simulink model "current_senzor"  (R2026a)
settings: Solver=VariableStepAuto
libraries: fl_lib x1, nesl_utility x1
settings Model: Creator=Fer Alexandru  LastModifiedBy=Fer Alexandru

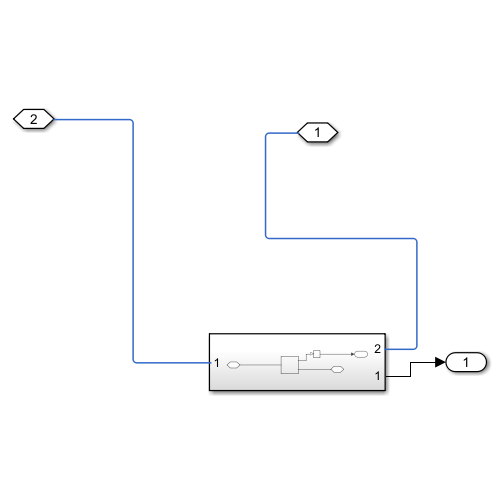
[thumbnail: Simulink's stored preview of the top-level diagram]
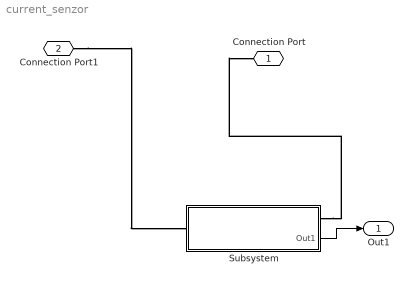
== system current_senzor ==
  Subsystem : Subsystem
      settings: PortSchema="{\"entries\":[{\"content\":{\"sides\":[{\"content\":{\"connectorIds\":[\"LConn1\"]},\"type\":\"ConnectorPlacement.EquallySpacedRectSide\",\"uuid\":\"879ab8e1-2049-4fb6-a8df-ff1276883f7d\"},{\"content\":{\"connectorIds\":[\"RConn1\",\"Out1\"],\"side\":\"RIGHT\"},\"type\":\"ConnectorPlacement.EquallySpacedRectSide\",\"uuid\":\"0e1e5d09-9c15-402d-9d9c-86393e5954a8\"},{\"content\":{\"side\":\"TOP\"},\"type\":\"ConnectorPlacement.EquallySpacedRectSide\",\"uuid\":\"a34ce212-58b0-488c-a820-7ab63fbdabb5\"}]},\"type\":\"ConnectorPlacement.EquallySpacedConnector\",\"uuid\":\"d04d41d3-98ba-4b02-a4fb-520314011242\"}],\"packageUris\":[\"http://schema.mathworks.com/mf0/Connector/R2020b\"],\"version\":\"1.0\"}"
  Connection Port : PMIOPort  Side=Left
  Connection Port1 : PMIOPort  Port=2  Side=Left
  Out1 : Outport
  wires:
  Subsystem/1(Out1) -> Out1/1
  connections:
  Subsystem/RConn1 -- Connection Port/RConn1
  Connection Port1/RConn1 -- Subsystem/LConn1

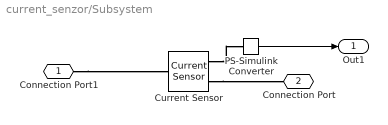
== system current_senzor/Subsystem ==
  Current Sensor : fl_lib/Electrical/Electrical Sensors/Current Sensor
  PS-Simulink Converter : nesl_utility/PS-Simulink Converter  PhysicalDomain=network_engine_domain  SubClassName=ps_output  LeftPortType=input  RightPortType=output  PseudoPeriodic=off  Frequencies=[]  VectorFormat=inherit  Unit=inherit  AffineConversion=off
  Connection Port1 : PMIOPort  Side=Left
  Connection Port : PMIOPort  Port=2  Side=Right
  Out1 : Outport
  wires:
  PS-Simulink Converter/1 -> Out1/1
  connections:
  Connection Port1/RConn1 -- Current Sensor/LConn1
  Current Sensor/RConn1 -- PS-Simulink Converter/LConn1
  Current Sensor/RConn2 -- Connection Port/RConn1
